simulink model "Analog_Irrigation_Control_System"  (R2026a)
settings: Solver=ode45  StopTime=60  MaxStep=0.001
undefined symbols (not defined in the file or in its folder): DiscIntNeverNeededParam
libraries: simulink x1
settings Model: Creator=hites  LastModifiedBy=hites
settings DataIOCC: OutputSaveName=vout

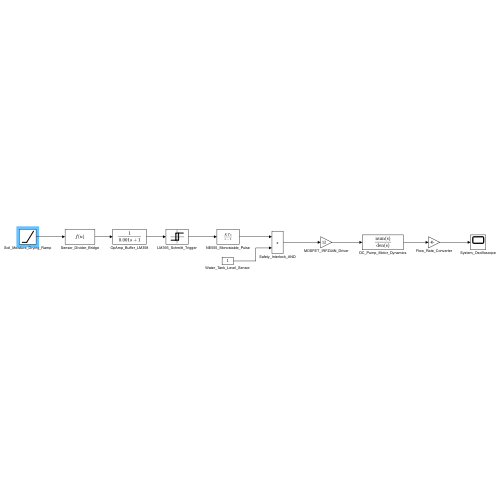
[thumbnail: Simulink's stored preview of the top-level diagram]
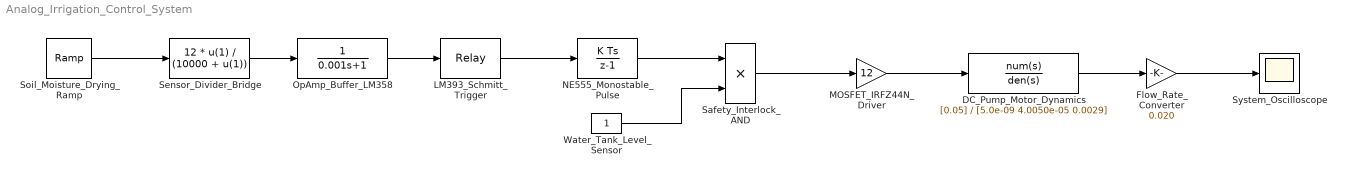
== system Analog_Irrigation_Control_System ==
  DC_Pump_Motor_Dynamics : TransferFcn  Numerator=[0.05]  Denominator=[5.0e-09 4.0050e-05 0.0029]
  Flow_Rate_Converter : Gain  Gain=0.020
  LM393_Schmitt_Trigger : Relay  OnSwitchValue=3.36  OffSwitchValue=2.27
  MOSFET_IRFZ44N_Driver : Gain  Gain=12
  NE555_Monostable_Pulse : DiscreteIntegrator  SampleTime=0.01  ICPrevOutput=DiscIntNeverNeededParam  ICPrevScaledInput=DiscIntNeverNeededParam
  OpAmp_Buffer_LM358 : TransferFcn  Denominator=[0.001 1]
  Safety_Interlock_AND : Product
  Sensor_Divider_Bridge : Fcn  Expr=12 * u(1) / (10000 + u(1))
  Soil_Moisture_Drying_Ramp : simulink/Sources/Ramp  slope=2000  start=5  InitialOutput=10000
  System_Oscilloscope : Scope
      settings: ActiveDisplayYMinimum=-31.019290067301693  ActiveDisplayYMaximum=279.17361060571528
  Water_Tank_Level_Sensor : Constant
  wires:
  OpAmp_Buffer_LM358/1 -> LM393_Schmitt_Trigger/1
  Safety_Interlock_AND/1 -> MOSFET_IRFZ44N_Driver/1
  Sensor_Divider_Bridge/1 -> OpAmp_Buffer_LM358/1
  Soil_Moisture_Drying_Ramp/1 -> Sensor_Divider_Bridge/1
  MOSFET_IRFZ44N_Driver/1 -> DC_Pump_Motor_Dynamics/1
  NE555_Monostable_Pulse/1 -> Safety_Interlock_AND/1
  LM393_Schmitt_Trigger/1 -> NE555_Monostable_Pulse/1
  Water_Tank_Level_Sensor/1 -> Safety_Interlock_AND/2
  DC_Pump_Motor_Dynamics/1 -> Flow_Rate_Converter/1
  Flow_Rate_Converter/1 -> System_Oscilloscope/1
